simulink model "Flicker_Noise"  (R2024a)
settings: Solver=VariableStepAuto  StartTime=0.0  StopTime=1  RelTol=1e-3
undefined symbols (not defined in the file): dspblkCoreblockFVToolHelper, gcbh
libraries: simulink_extras x2, cstblocks x1, dspobslib x1, dspsigops x1
settings Model: Creator=Hp  LastModifiedBy=Hp

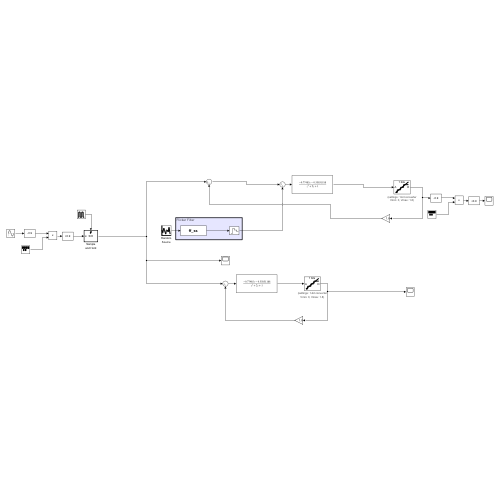
[thumbnail: Simulink's stored preview of the top-level diagram]
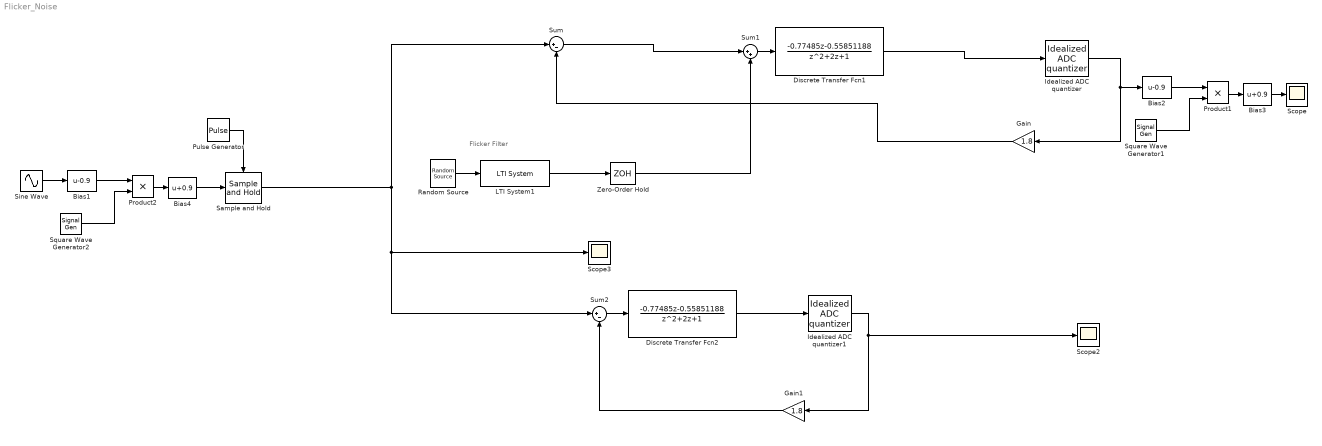
== system Flicker_Noise ==
  note: Flicker Filter
  Bias1 : Bias  Bias=-0.9  SaturateOnIntegerOverflow=off
  Bias2 : Bias  Bias=-0.9  SaturateOnIntegerOverflow=off
  Bias3 : Bias  Bias=0.9  SaturateOnIntegerOverflow=off
  Bias4 : Bias  Bias=0.9  SaturateOnIntegerOverflow=off
  Discrete Transfer Fcn1 : DiscreteTransferFcn  LoadFcn=dspblkCoreblockFVToolHelper(gcbh,'load');  Numerator=[-0.77485 -0.55851188]  Denominator=[1 +2 1]
      settings: CopyFcn=dspblkCoreblockFVToolHelper(gcbh,'copy');  DeleteFcn=dspblkCoreblockFVToolHelper(gcbh,'close');  ModelCloseFcn=dspblkCoreblockFVToolHelper(gcbh,'close');  PreSaveFcn=dspblkCoreblockFVToolHelper(gcbh,'presave');  PostSaveFcn=dspblkCoreblockFVToolHelper(gcbh,'postsave');  CloseFcn=dspblkCoreblockFVToolHelper(gcbh,'close');
  Discrete Transfer Fcn2 : DiscreteTransferFcn  LoadFcn=dspblkCoreblockFVToolHelper(gcbh,'load');  Numerator=[-0.77485 -0.55851188]  Denominator=[1 +2 1]
      settings: CopyFcn=dspblkCoreblockFVToolHelper(gcbh,'copy');  DeleteFcn=dspblkCoreblockFVToolHelper(gcbh,'close');  ModelCloseFcn=dspblkCoreblockFVToolHelper(gcbh,'close');  PreSaveFcn=dspblkCoreblockFVToolHelper(gcbh,'presave');  PostSaveFcn=dspblkCoreblockFVToolHelper(gcbh,'postsave');  CloseFcn=dspblkCoreblockFVToolHelper(gcbh,'close');
  Gain : Gain  Gain=1.8
  Gain1 : Gain  Gain=1.8
  Idealized ADC quantizer : simulink_extras/Additional Discrete/Idealized ADC quantizer  NumberOfConverterBits=1  Vmin=0  Vmax=1.8  OutputDataType=int32  OutputNegativeValues=off
  Idealized ADC quantizer1 : simulink_extras/Additional Discrete/Idealized ADC quantizer  NumberOfConverterBits=1  Vmin=0  Vmax=1.8  OutputDataType=int32  OutputNegativeValues=off
  LTI System1 : cstblocks/LTI System  sys=ff_ss  IC=[]  PadeOrder=0
  Product1 : Product
  Product2 : Product
  Pulse Generator : DiscretePulseGenerator  PulseType=Time based  Period=1/2048000  PulseWidth=50
  Random Source : dspobslib/Random Source  SrcType=Gaussian  NormMethod=Ziggurat  CltLength=12  MinVal=0  MaxVal=1  MeanVal=0  VarVal=1e-8  RepMode=Not repeatable  rawSeed=1  IsInherit=off  SampMode=Discrete  SampTime=1/(2000*1024)  SampFrame=1  DataType=Double  OutComplex=Real  OutputFrames=off
  Sample and Hold : dspsigops/Sample and Hold  trig=Rising edge  initCond=0  latchinput=off
  Scope : Scope
  Scope2 : Scope
  Scope3 : Scope
  Sine Wave : Sin  Amplitude=0.5  Bias=0.9  Frequency=((2000*1024)*127*2*2*pi)/(32768*32)  SampleTime=0
  Square Wave Generator1 : SignalGenerator  WaveForm=square  Frequency=2048000/2
  Square Wave Generator2 : SignalGenerator  WaveForm=square  Frequency=2048000/2
  Sum : Sum  Inputs=|+-
  Sum1 : Sum  Inputs=|++
  Sum2 : Sum  Inputs=|+-
  Zero-Order Hold : ZeroOrderHold  SampleTime=1/(2000*1024)
  wires:
  Sample and Hold/1 -> Sum/1, Scope3/1, Sum2/1
  Gain/1 -> Sum/2
  Random Source/1 -> LTI System1/1
  LTI System1/1 -> Zero-Order Hold/1
  Gain1/1 -> Sum2/2
  Discrete Transfer Fcn2/1 -> Idealized ADC quantizer1/1
  Sum2/1 -> Discrete Transfer Fcn2/1
  Idealized ADC quantizer1/1 -> Gain1/1, Scope2/1
  Zero-Order Hold/1 -> Sum1/2
  Sum1/1 -> Discrete Transfer Fcn1/1
  Discrete Transfer Fcn1/1 -> Idealized ADC quantizer/1
  Sum/1 -> Sum1/1
  Square Wave Generator1/1 -> Product1/2
  Idealized ADC quantizer/1 -> Bias2/1, Gain/1
  Product1/1 -> Bias3/1
  Bias2/1 -> Product1/1
  Bias3/1 -> Scope/1
  Sine Wave/1 -> Bias1/1
  Square Wave Generator2/1 -> Product2/2
  Product2/1 -> Bias4/1
  Bias1/1 -> Product2/1
  Bias4/1 -> Sample and Hold/1
  Pulse Generator/1 -> Sample and Hold/Trigger
